simulink model "cogging_comp_AFC_2026_0910"  (R2019a)
settings: Solver=FixedStepDiscrete  StartTime=0.0  StopTime=880  FixedStep=0.001  RelTol=1e-3  EnableMultiTasking=on
undefined symbols (not defined in the file): DiscIntNeverNeededParam, Tcog, Tcog_15
libraries: sbox2 x4, simulink x1, dspsigops x1
settings Model: Creator=haketa  LastModifiedBy=アクチュエータダンパ班
settings DataIOCC: LimitDataPoints=on  SaveFormat=Array  ReturnWorkspaceOutputs=off
settings OptimizationCC: BlockReduction=off  OptimizeBlockIOStorage=off  BufferReuse=off  GlobalBufferReuse=off  ExpressionFolding=off  ExpressionDepthLimit=2147483647  LocalBlockOutputs=off  InitFltsAndDblsToZero=on  LifeSpan=inf  OptimizeDataStoreBuffers=off  BusAssignmentInplaceUpdate=off
settings DebuggingCC: SaveWithParameterizedLinksMsg=none  UnderspecifiedInitializationDetection=Classic  MergeDetectMultiDrivingBlocksExec=none  SignalResolutionControl=TryResolveAllWithWarning  SolverPrmCheckMsg=warning  InheritedTsInSrcMsg=none  MultiTaskDSMMsg=warning  MultiTaskCondExecSysMsg=none  FcnCallInpInsideContextMsg=warning  StateNameClashWarn=warning  SFUnexpectedBacktrackingDiag=warning  SFNoUnconditionalDefaultTransitionDiag=warning  SFExecutionAtInitializationDiag=none  ArithmeticOperatorsInVariantConditions=warning
settings HardwareCC: ProdBitPerPointer=32  ProdBitPerSizeT=32  ProdBitPerPtrDiffT=32  ProdLargestAtomicFloat=None  ProdIntDivRoundTo=Undefined  ProdEndianess=Unspecified  ProdWordSize=32  ProdHWDeviceType=32-bit Generic
settings ModelReferenceCC: PropagateSignalLabelsOutOfModel=off
settings SFSimCC: SimUseLocalCustomCode=off
settings RTWCC: SystemTargetFile=sbox2.tlc  TemplateMakefile=sbox2.tmf  Description=MTT sBOXII Real-Time Target.  RTWUseLocalCustomCode=off  RTWCompilerOptimization=on
settings CodeAppCC: StateflowObjectComments=on
settings GRTTargetCC: TargetLangStandard=C89/C90 (ANSI)  GeneratePreprocessorConditionals=Disable all  MatFileLogging=off  UseToolchainInfoCompliant=off  RTWCAPISignals=on  RTWCAPIParams=on
settings ConfigComp: CovMetricSettings=dw  CovHtmlReporting=on  CovSaveCumulativeToWorkspaceVar=on  CovSaveSingleToWorkspaceVar=on  CovExternalEMLEnable=off  CovSFcnEnable=off

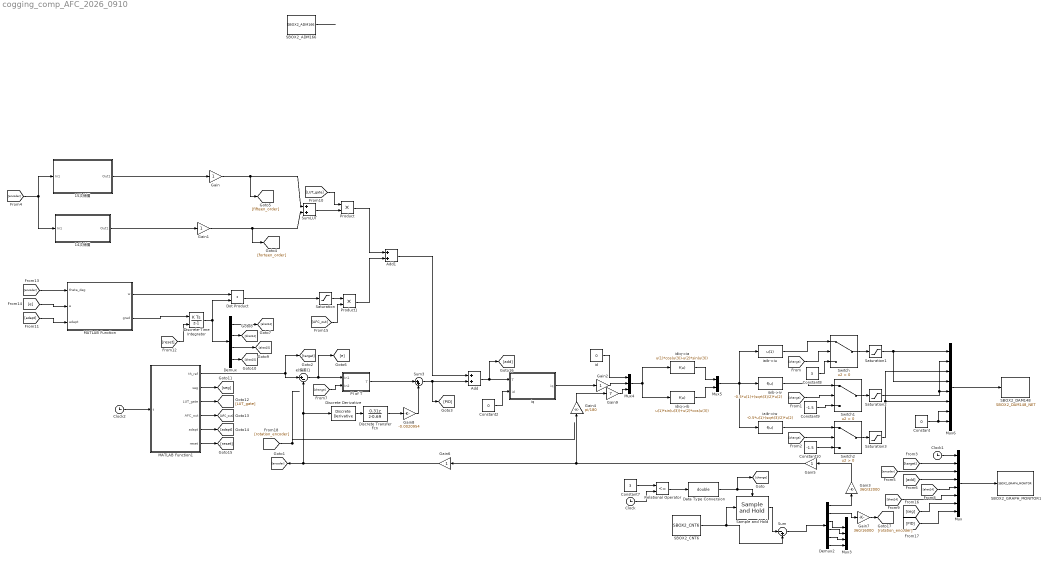
== system cogging_comp_AFC_2026_0910 ==
  14次補償 : Subsystem
  15次補償 : Subsystem
  Add : Sum
  Add1 : Sum
  Clock : Clock
  Clock1 : Clock
  Clock2 : Clock
  Constant : Constant  Value=0
  Constant10 : Constant  Value=-1.5
  Constant2 : Constant  Value=0
  Constant7 : Constant  Value=3
  Constant8 : Constant  Value=3
  Constant9 : Constant  Value=-1.5
  Data Type Conversion : DataTypeConversion  OutDataTypeStr=double
  Demux : Demux
  Demux2 : Demux  Outputs=6
  Discrete Transfer Fcn : DiscreteTransferFcn  Numerator=[0.31 0]  Denominator=[1 -0.69]
  Discrete Derivative : simulink/Discrete/Discrete Derivative  gainval=1.0  ICPrevScaledInput=0.0  OutMin=[]  OutMax=[]  OutDataType=fixdt(1, 16)  OutScaling=2^-10  DoSatur=off
  Discrete-Time Integrator : DiscreteIntegrator  ExternalReset=rising  SampleTime=-1  ICPrevOutput=DiscIntNeverNeededParam  ICPrevScaledInput=DiscIntNeverNeededParam
  Dot Product : DotProduct  InputSameDT=on  OutDataTypeStr=Inherit: Inherit via internal rule
  Gain{,1..2,5..6} (5 alike) : Gain
  Gain3 : Gain  Gain=360/32000
  Gain4 : Gain  Gain=pi/180
  Gain7 : Gain  Gain=360/16000
  Gain8 : Gain  Gain=-0.0020954
  Gain9 : Gain  Gain=7
  MATLAB Function : MATLAB Function  TreatAsAtomicUnit=on
  MATLAB Function1 : MATLAB Function  TreatAsAtomicUnit=on
  Mux : Mux  Inputs=8
  Mux3 : Mux  Inputs=5
  Mux4 : Mux  Inputs=3
  Mux5 : Mux  Inputs=2
  Mux6 : Mux  Inputs=8
  PI of T : Subsystem
  Product : Product
  Product1 : Product
  Relational Operator : RelationalOperator  Operator=<=  OutDataTypeStr=boolean  RndMeth=Simplest
  SBOX2_ADM166 : sbox2/Analog I//O Devices/SBOX2_ADM166  sampletime=-1
  SBOX2_CNT6 : sbox2/Digital I//O Devices/SBOX2_CNT6  mode=2相パルス  teibai=x4  filter=off  zphase=動作なし  polarity=正論理 (high active)  mode2=2相パルス  teibai2=x4  filter2=off  zphase2=動作なし  polarity2=正論理 (high active)  mode3=2相パルス  teibai3=x4  filter3=off  zphase3=動作なし  polarity3=正論理 (high active)  mode4=2相パルス  teibai4=x4  filter4=off  zphase4=動作なし  polarity4=正論理 (high active)  mode5=2相パルス  teibai5=x4  filter5=off  zphase5=動作なし  polarity5=正論理 (high active)  mode6=2相パルス  teibai6=x4  filter6=off  zphase6=動作なし  polarity6=正論理 (high active)  dtype=FLOATING POINT  sampletime=-1
  "SBOX2_DAM148 " : sbox2/Analog I//O Devices/SBOX2_DAM148_NET  daStopCtrl1=0V出力  daStopCtrl2=DA出力継続  daStopCtrl3=DA出力継続  daStopCtrl4=DA出力継続  daStopCtrl5=DA出力継続  daStopCtrl6=DA出力継続  daStopCtrl7=DA出力継続  daStopCtrl8=DA出力継続  sampletime=-1
  SBOX2_GRAPH_MONITOR1 : sbox2/Network Data Save Devices/SBOX2_GRAPH_MONITOR  sampletime=-1
  Sample and Hold : dspsigops/Sample and Hold  trig=Rising edge  initCond=0  latchinput=off
  Saturation{,1..3} (4 alike) : Saturate  UpperLimit=5  LowerLimit=-5
  Sum : Sum  Inputs=|-+
  Sum3 : Sum  Inputs=|++
  SumLUT : Sum
  Switch : Switch  Criteria=u2 > Threshold
  Switch1 : Switch  Criteria=u2 > Threshold
  Switch2 : Switch  Criteria=u2 > Threshold
  e(偏差)1 : Sum  Inputs=|+-
  iaib->iu : Fcn  Expr=u(1)
  iaib->iv : Fcn  Expr=-0.5*u(1)+(sqrt(3)/2)*u(2)
  iaib->iw : Fcn  Expr=-0.5*u(1)-(sqrt(3)/2)*u(2)
  id : Constant  Value=0
  idiq->ia : Fcn  Expr=u(1)*cos(u(3))-u(2)*sin(u(3))
  idiq->ib : Fcn  Expr=u(1)*sin(u(3))+u(2)*cos(u(3))
  iq : MATLAB Function  TreatAsAtomicUnit=on
  wires:
  SBOX2_ADM166/1 -> ?
  Relational Operator/1 -> Data Type Conversion/1
  Clock/1 -> Relational Operator/2
  [change] -> Switch/2
  iaib->iw/1 -> Switch2/1
  Demux2/6 -> Mux3/5
  SBOX2_CNT6/1 -> Sample and Hold/1, Sum/2
  Constant7/1 -> Relational Operator/1
  Gain2/1 -> Mux4/2
  Gain3/1 -> Gain5/1
  Add/1 -> [add], iq/1(T)
  Sum/1 -> Demux2/1
  Demux2/4 -> Mux3/3
  Demux2/3 -> Mux3/2
  Gain6/1 -> [encoder], Discrete Derivative/1, e(偏差)1/2
  Mux6/1 -> "SBOX2_DAM148 "/1
  e(偏差)1/1 -> [e], PI of T/1(In1)
  Gain8/1 -> Sum3/2
  Mux5/1 -> iaib->iw/1, iaib->iv/1, iaib->iu/1
  Sample and Hold/1 -> Sum/1
  Constant9/1 -> Switch1/3
  iq/1(iq) -> Gain2/1
  id/1 -> Mux4/1
  Discrete Derivative/1 -> Discrete Transfer Fcn/1
  Gain4/1 -> Gain9/1
  Constant2/1 -> iq/2(id)
  Switch/1 -> Saturation1/1
  Constant8/1 -> Switch/3
  PI of T/1(T) -> Sum3/1
  Mux4/1 -> idiq->ib/1, idiq->ia/1
  iaib->iu/1 -> Switch/1
  Saturation3/1 -> Mux6/3, Mux6/6
  Gain5/1 -> Gain4/1, Gain6/1
  Switch2/1 -> Saturation3/1
  Saturation2/1 -> Mux6/2, Mux6/5
  iaib->iv/1 -> Switch1/1
  Sum3/1 -> Add/2, [PID]
  Saturation1/1 -> Mux6/1, Mux6/4
  Demux2/1 -> Gain3/1
  Data Type Conversion/1 -> [change], Sample and Hold/Trigger
  idiq->ia/1 -> Mux5/1
  idiq->ib/1 -> Mux5/2
  [change] -> Switch1/2
  Discrete Transfer Fcn/1 -> Gain8/1
  Switch1/1 -> Saturation2/1
  [change] -> Switch2/2
  Gain9/1 -> Mux4/3
  Demux2/5 -> Mux3/4
  Constant10/1 -> Switch2/3
  MATLAB Function1/1(th_ref) -> e(偏差)1/1, [target]
  Gain/1 -> [fifteen_order], SumLUT/1
  14次補償/1(Out1) -> Gain1/1
  15次補償/1(Out1) -> Gain/1
  [encoder] -> 15次補償/1(In1), 14次補償/1(In1)
  Gain1/1 -> SumLUT/2, [forteen_order]
  Constant/1 -> Mux6/7, Mux6/8
  Mux/1 -> SBOX2_GRAPH_MONITOR1/1
  Clock1/1 -> Mux/1
  [target] -> Mux/2
  [encoder] -> Mux/3
  [add] -> Mux/4
  [change] -> PI of T/2(In2)
  [ahat14] -> Mux/5
  [bhat14] -> Mux/6
  SumLUT/1 -> Product/2
  [LUT_gate] -> Product/1
  [encoder] -> MATLAB Function/1(theta_deg)
  [e] -> MATLAB Function/2(e)
  Dot Product/1 -> Saturation/1
  [AFC_out] -> Product1/2
  Product/1 -> Add1/1
  Product1/1 -> Add1/2
  Add1/1 -> Add/1
  Saturation/1 -> Product1/1
  MATLAB Function/1(w) -> Dot Product/1
  MATLAB Function/2(grad) -> Discrete-Time Integrator/1
  Discrete-Time Integrator/1 -> Demux/1, Dot Product/2
  Demux/4 -> [bhat15]
  Demux/3 -> [ahat15]
  Demux/2 -> [bhat14]
  Demux/1 -> [ahat14]
  Clock2/1 -> MATLAB Function1/1(t)
  MATLAB Function1/2(seg) -> [seg]
  MATLAB Function1/3(LUT_gate) -> [LUT_gate]
  MATLAB Function1/4(AFC_out) -> [AFC_out]
  MATLAB Function1/5(adapt) -> [adapt]
  MATLAB Function1/6(reset) -> [reset]
  [adapt] -> MATLAB Function/3(adapt)
  [reset] -> Discrete-Time Integrator/2
  [seg] -> Mux/7
  [PID] -> Mux/8
  Gain7/1 -> [rotation_encoder]
  Demux2/2 -> Gain7/1
  [rotation_encoder] -> ?

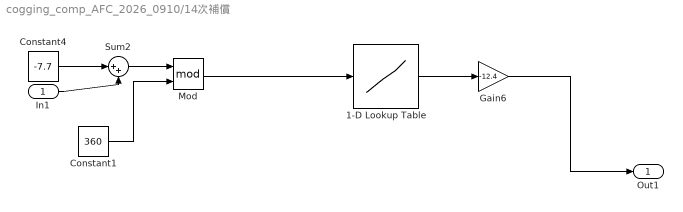
== system cogging_comp_AFC_2026_0910/14次補償 ==
  In1 : Inport
  1-D Lookup Table : Lookup_n-D  NumberOfTableDimensions=1  BreakpointsForDimension1=angle  Table=Tcog  InterpMethod=Cubic spline  ExtrapMethod=Cubic spline  InternalRulePriority=Speed  RndMeth=Simplest  InputSameDT=on
  Constant1 : Constant  Value=360
  Constant4 : Constant  Value=-7.7
  Gain6 : Gain  Gain=-12.4
  Mod : Math  Operator=mod  SaturateOnIntegerOverflow=on
  Sum2 : Sum  Inputs=|++
  Out1 : Outport
  wires:
  Mod/1 -> 1-D Lookup Table/1
  Gain6/1 -> Out1/1
  1-D Lookup Table/1 -> Gain6/1
  Constant1/1 -> Mod/2
  In1/1 -> Sum2/2
  Constant4/1 -> Sum2/1
  Sum2/1 -> Mod/1

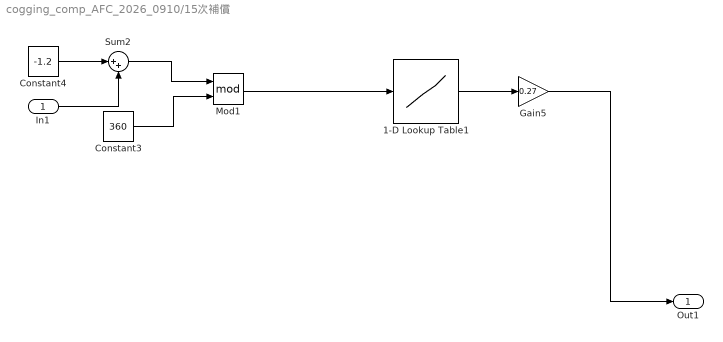
== system cogging_comp_AFC_2026_0910/15次補償 ==
  In1 : Inport
  1-D Lookup Table1 : Lookup_n-D  NumberOfTableDimensions=1  BreakpointsForDimension1=angle  Table=Tcog_15  InterpMethod=Cubic spline  ExtrapMethod=Cubic spline  InternalRulePriority=Speed  RndMeth=Simplest  InputSameDT=on
  Constant3 : Constant  Value=360
  Constant4 : Constant  Value=-1.2
  Gain5 : Gain  Gain=0.27
  Mod1 : Math  Operator=mod  SaturateOnIntegerOverflow=on
  Sum2 : Sum  Inputs=|++
  Out1 : Outport
  wires:
  Mod1/1 -> 1-D Lookup Table1/1
  Constant3/1 -> Mod1/2
  1-D Lookup Table1/1 -> Gain5/1
  In1/1 -> Sum2/2
  Gain5/1 -> Out1/1
  Constant4/1 -> Sum2/1
  Sum2/1 -> Mod1/1

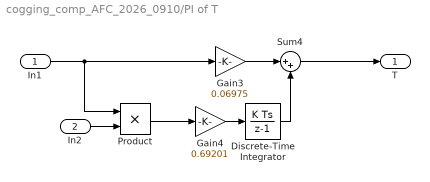
== system cogging_comp_AFC_2026_0910/PI of T ==
  In1 : Inport
  In2 : Inport  Port=2
  Discrete-Time Integrator : DiscreteIntegrator  SampleTime=-1  ICPrevOutput=DiscIntNeverNeededParam  ICPrevScaledInput=DiscIntNeverNeededParam
  Gain3 : Gain  Gain=0.06975
  Gain4 : Gain  Gain=0.69201
  Product : Product
  Sum4 : Sum  Inputs=|++
  T : Outport  VectorParamsAs1DForOutWhenUnconnected=on
  wires:
  In1/1 -> Product/1, Gain3/1
  Discrete-Time Integrator/1 -> Sum4/2
  Gain4/1 -> Discrete-Time Integrator/1
  Sum4/1 -> T/1
  Gain3/1 -> Sum4/1
  Product/1 -> Gain4/1
  In2/1 -> Product/2

== matlab function cogging_comp_AFC_2026_0910/MATLAB Function ==
  data: theta_deg input; w output; grad output; e input; adapt input
function [w, grad] = afc_core(theta_deg, e, adapt)
%#codegen
% ===== 設定　次数を増やす時は3行とも要素を足す =====
N   = [14,     15    ];   % 次数
G   = [0.02,  0.02   ];   % 適応外院g_n  [N*m/(deg*s)]
PHI = [0.0, 0.0   ];   % 位相進み phi_n  [rad]  
% ====================================================

M    = numel(N);
w    = zeros(2*M, 1);
grad = zeros(2*M, 1);

for k = 1:M
    psi = mod(N(k)*theta_deg, 360) * pi/180;   % 0～2pi [rad]

    w(2*k-1) = cos(psi);
    w(2*k  ) = sin(psi);

    a = G(k) * e * adapt;
    grad(2*k-1) = a * cos(psi + PHI(k));
    grad(2*k  ) = a * sin(psi + PHI(k));
end
end

== matlab function cogging_comp_AFC_2026_0910/iq ==
  data: T input; iq output; id input
function iq = fcn(T, id)

% ==== パラメータ（必要に応じて変更） ====
p = 7;              % 極対数
psi_f = 0.107;       % 永久磁石磁束 [Wb]
Ld = 11.2*10^-3;         % d軸インダクタンス [H]
Lq = 19*10^-3;         % q軸インダクタンス [H]

% ==== 計算 ====
den = (3/2)*p * (psi_f + (Ld - Lq)*id);
iq = T / den;

% % 0割り防止
% if abs(den) < 1e-6
%     iq = 0;
% else
%     iq = T / den;
end

== matlab function cogging_comp_AFC_2026_0910/MATLAB Function1 ==
  data: t input; th_ref output; seg output; LUT_gate output; AFC_out output; adapt output; reset output
function [th_ref, seg, LUT_gate, AFC_out, adapt, reset] = sched(t)
%#codegen
% =============== 実行ごとに変えるのはここのみ ===============
OMG = 5.157;   % [deg/s]
%   5.157 = 0.09 rad/s   StopTime 879
%   8.594 = 0.15         StopTime 531
%  14.324 = 0.25         StopTime 325
%  22.918 = 0.40         StopTime 241
%  34.377 = 0.60         StopTime 218
%  51.566 = 0.90         StopTime 217
% =============================================================
T0 = 5.0;

% --- 速度ごとの区間長（w=解析窓，L＝学習）---
if     OMG <  7,   W = 140;  L = 439;
elseif OMG < 11,   W =  84;  L = 259;
elseif OMG < 18,   W =  50;  L = 155;
elseif OMG < 28,   W =  40;  L = 101;
elseif OMG < 42,   W =  40;  L =  78;
else               W =  40;  L =  77;
end

t1 = 20;   t2 = t1 + W;   t3 = t2 + L;   t4 = t3 + W;   t5 = t4 + W;
t6 = t5 + L; t7 = t6 + W;

th_ref = 0; seg = 0; LUT_gate = 0; AFC_out = 0; adapt = 0; reset = 0;

if t >= T0
    th_ref = OMG * (t - T0);
end

if     t < t1,  seg = 0;                             % settle
elseif t < t2,  seg = 2;                             % baseline
elseif t < t3,  seg = 3;  AFC_out = 1;  adapt = 1;   % learning
elseif t < t4,  seg = 4;  AFC_out = 1;               % frozen
elseif t < t5,  seg = 5;  LUT_gate = 1;              % LUT only
elseif t < t6,  seg = 6;  LUT_gate = 1; AFC_out = 1; adapt = 1; %LUT, AFC併用　学習期間
elseif t < t7,  seg = 7;  LUT_gate = 1; AFC_out = 1; % LUT，AFC併用・凍結
else            seg = 9;
end

if (t >= t2 && t < t2 + 0.0015) || (t >= t5 && t < t5 + 0.0015)
    reset = 1;
end

adapt = adapt * AFC_out;
end
